simulink model "bins_model2"  (Simulink 8.3)
settings: Solver=ode45  StartTime=0.0  StopTime=300  MaxStep=0.1  RelTol=1e-3
libraries: aerolibnav x1
settings Model: Creator=me  LastModifiedBy=me
settings DataIOCC: SignalLoggingSaveFormat=Dataset
settings DebuggingCC: UnderspecifiedInitializationDetection=Simplified  StateNameClashWarn=none
settings GRTTargetCC: CombineOutputUpdateFcns=on  GRTInterface=off

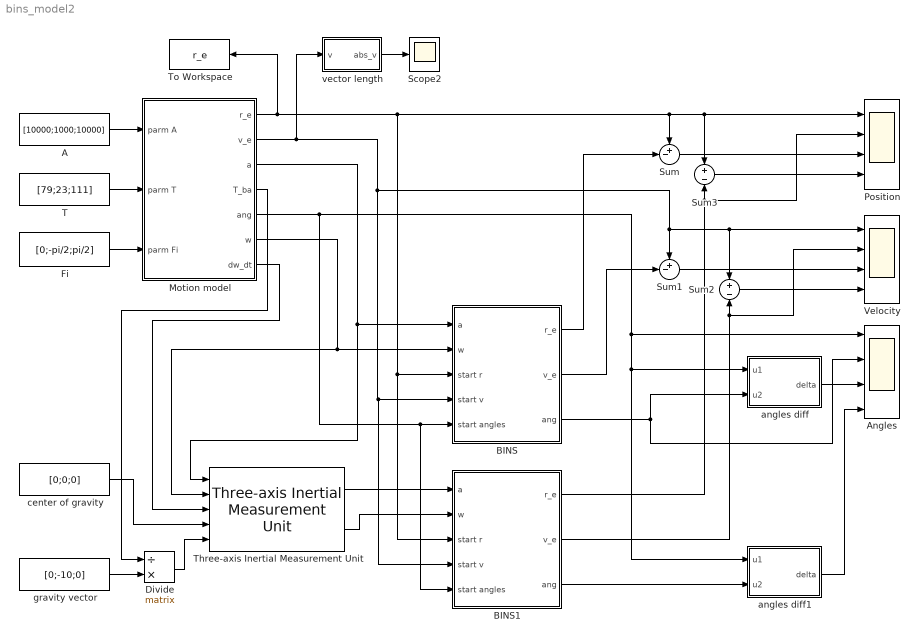
== system bins_model2 ==
  A : Constant  Value=[10000;1000;10000]
  Angles : Scope  NumInputPorts=4
      settings: TimeRange=300  YMin=-4~-4~-3e-15~-7  YMax=4~4~4e-15~1  SaveName=ScopeData3  MaxDataPoints=200000
  BINS : Subsystem
  BINS1 : Subsystem
  Divide : Product  Inputs=/*  Multiplication=Matrix(*)
  Fi : Constant  Value=[0;-pi/2;pi/2]
  Motion model : Subsystem
  Position : Scope  NumInputPorts=4
      settings: TimeRange=300  YMin=-10000~-20000~-1e-09~-10000  YMax=10000~20000~3e-09~5000  MaxDataPoints=200000
  Scope2 : Scope
      settings: TimeRange=1000  YMin=0  YMax=1000  SaveName=ScopeData2  MaxDataPoints=50000
  Sum : Sum  Inputs=+-|
  Sum1 : Sum  Inputs=+-|
  Sum2 : Sum  Inputs=+-
  Sum3 : Sum  Inputs=+-
  T : Constant  Value=[79;23;111]
  Three-axis Inertial Measurement Unit : aerolibnav/Three-axis Inertial Measurement Unit  units=Metric (MKS)  imu=[0 0 0]  dtype_a=off  w_a=190  z_a=0.707  a_sf_cc=[1 0 0; 0 1 0; 0 0 1]  a_bias=[0 0 0]  a_sat="[-inf  -inf  -inf  inf inf inf]"  dtype_g=off  w_g=190  z_g=0.707  g_sf_cc=[1 0 0; 0 1 0; 0 0 1]  g_bias=[0 0 0]  g_sens=[0 0 0]  g_sat="[-inf  -inf  -inf  inf inf inf]"  i_rand=on  i_seeds=[23093 23094 23095 23096 23097 23098]  i_pow=[0.0001 0.0001 0.0001 0.000001 0.000001 0.000001]  i_Ts=0
  To Workspace : ToWorkspace  VariableName=r_e  SaveFormat=Timeseries  SampleTime=-1
  Velocity : Scope  NumInputPorts=4
      settings: TimeRange=1000  YMin=-1000~-1000~-1e-09~-100  YMax=1000~1000~1e-09~100  SaveName=ScopeData4  MaxDataPoints=200000
  angles diff : MATLAB Function  TreatAsAtomicUnit=on
  angles diff1 : MATLAB Function  TreatAsAtomicUnit=on
  center of gravity : Constant  Value=[0;0;0]
  gravity vector : Constant  Value=[0;-10;0]
  vector length : Subsystem
  wires:
  vector length/1(abs_v) -> Scope2/1
  A/1 -> Motion model/1(parm A)
  T/1 -> Motion model/2(parm T)
  Fi/1 -> Motion model/3(parm Fi)
  Motion model/1(r_e) -> BINS1/3(start r), BINS/3(start r), Sum/1, Position/1, Sum3/1, To Workspace/1
  Motion model/5(ang) -> BINS1/5(start angles), BINS/5(start angles), angles diff1/1(u1), angles diff/1(u1), Angles/1
  Motion model/3(a) -> Three-axis Inertial Measurement Unit/1, BINS/1(a)
  Motion model/7(dw_dt) -> Three-axis Inertial Measurement Unit/3
  BINS/3(ang) -> angles diff/2(u2), Angles/2
  angles diff/1(delta) -> Angles/3
  BINS/1(r_e) -> Sum/2
  Sum/1 -> Position/3
  Motion model/2(v_e) -> BINS1/4(start v), BINS/4(start v), Sum1/1, Sum2/1, Velocity/1, vector length/1(v)
  BINS/2(v_e) -> Sum1/2
  Sum1/1 -> Velocity/3
  center of gravity/1 -> Three-axis Inertial Measurement Unit/4
  Three-axis Inertial Measurement Unit/1 -> BINS1/1(a)
  Three-axis Inertial Measurement Unit/2 -> BINS1/2("w ")
  Motion model/6(w) -> Three-axis Inertial Measurement Unit/2, BINS/2("w ")
  BINS1/3(ang) -> angles diff1/2(u2)
  angles diff1/1(delta) -> Angles/4
  Sum2/1 -> Velocity/4
  Sum3/1 -> Position/4
  BINS1/1(r_e) -> Position/2, Sum3/2
  BINS1/2(v_e) -> Velocity/2, Sum2/2
  gravity vector/1 -> Divide/2
  Divide/1 -> Three-axis Inertial Measurement Unit/5
  Motion model/4(T_ba) -> Divide/1

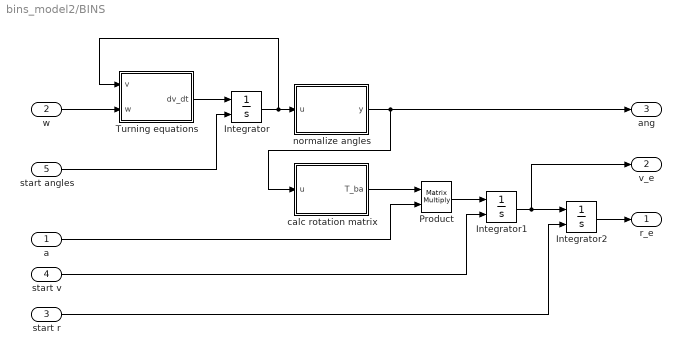
== system bins_model2/BINS ==
  a : Inport
  "w " : Inport  Port=2
  start r : Inport  Port=3
  start v : Inport  Port=4
  start angles : Inport  Port=5
  Integrator : Integrator  InitialConditionSource=external
  Integrator1 : Integrator  InitialConditionSource=external
  Integrator2 : Integrator  InitialConditionSource=external
  Product : Product  Multiplication=Matrix(*)
  Turning equations : MATLAB Function  TreatAsAtomicUnit=on
  calc rotation matrix : MATLAB Function  TreatAsAtomicUnit=on
  normalize angles : MATLAB Function  TreatAsAtomicUnit=on
  r_e : Outport
  v_e : Outport  Port=2
  ang : Outport  Port=3
  wires:
  Product/1 -> Integrator1/1
  Turning equations/1(dv_dt) -> Integrator/1
  Integrator/1 -> Turning equations/1(v), normalize angles/1(u)
  normalize angles/1(y) -> calc rotation matrix/1(u), ang/1
  Integrator1/1 -> Integrator2/1, v_e/1
  start r/1 -> Integrator2/2
  a/1 -> Product/2
  start v/1 -> Integrator1/2
  start angles/1 -> Integrator/2
  calc rotation matrix/1(T_ba) -> Product/1
  Integrator2/1 -> r_e/1
  "w "/1 -> Turning equations/2(w)

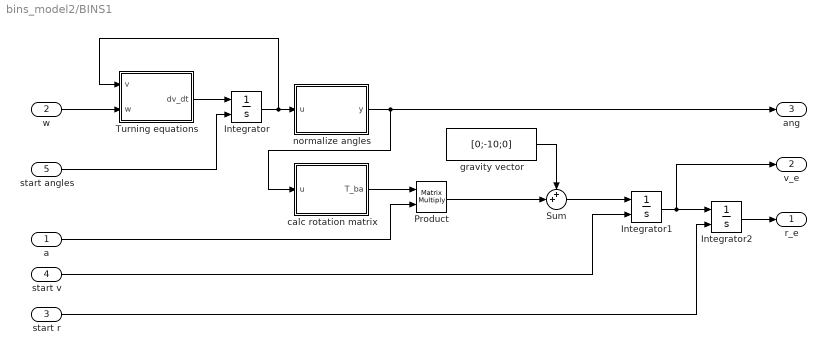
== system bins_model2/BINS1 ==
  a : Inport
  "w " : Inport  Port=2
  start r : Inport  Port=3
  start v : Inport  Port=4
  start angles : Inport  Port=5
  Integrator : Integrator  InitialConditionSource=external
  Integrator1 : Integrator  InitialConditionSource=external
  Integrator2 : Integrator  InitialConditionSource=external
  Product : Product  Multiplication=Matrix(*)
  Sum : Sum  Inputs=++|
  Turning equations : MATLAB Function  TreatAsAtomicUnit=on
  calc rotation matrix : MATLAB Function  TreatAsAtomicUnit=on
  gravity vector : Constant  Value=[0;-10;0]
  normalize angles : MATLAB Function  TreatAsAtomicUnit=on
  r_e : Outport
  v_e : Outport  Port=2
  ang : Outport  Port=3
  wires:
  Turning equations/1(dv_dt) -> Integrator/1
  Integrator/1 -> Turning equations/1(v), normalize angles/1(u)
  normalize angles/1(y) -> calc rotation matrix/1(u), ang/1
  Integrator1/1 -> Integrator2/1, v_e/1
  start r/1 -> Integrator2/2
  a/1 -> Product/2
  start angles/1 -> Integrator/2
  calc rotation matrix/1(T_ba) -> Product/1
  Integrator2/1 -> r_e/1
  "w "/1 -> Turning equations/2(w)
  gravity vector/1 -> Sum/1
  Sum/1 -> Integrator1/1
  Product/1 -> Sum/2
  start v/1 -> Integrator1/2

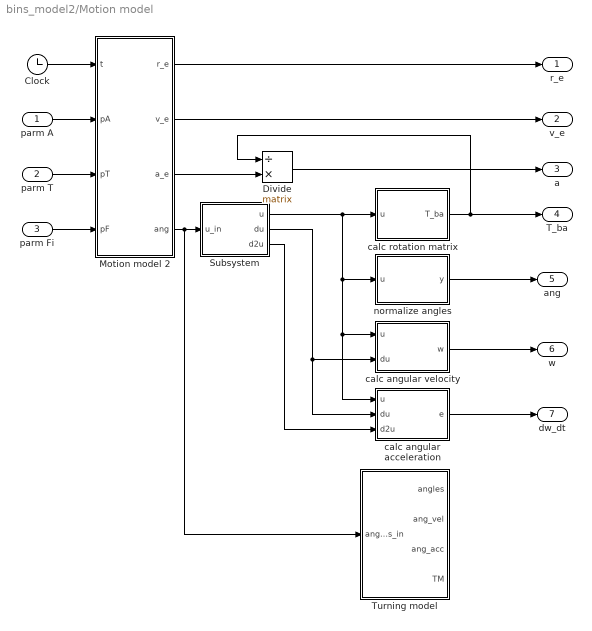
== system bins_model2/Motion model ==
  parm A : Inport
  parm T : Inport  Port=2
  parm Fi : Inport  Port=3
  Clock : Clock
  Divide : Product  Inputs=/*  Multiplication=Matrix(*)
  Motion model 2 : MATLAB Function  TreatAsAtomicUnit=on
  Subsystem : Subsystem
  Turning model : Subsystem
  calc angular acceleration : MATLAB Function  TreatAsAtomicUnit=on
  calc angular velocity : MATLAB Function  TreatAsAtomicUnit=on
  calc rotation matrix : MATLAB Function  TreatAsAtomicUnit=on
  normalize angles : MATLAB Function  TreatAsAtomicUnit=on
  r_e : Outport
  v_e : Outport  Port=2
  a : Outport  Port=3
  T_ba : Outport  Port=4
  ang : Outport  Port=5
  w : Outport  Port=6
  dw_dt : Outport  Port=7
  wires:
  parm Fi/1 -> Motion model 2/4(pF)
  parm A/1 -> Motion model 2/2(pA)
  parm T/1 -> Motion model 2/3(pT)
  Subsystem/2(du) -> calc angular acceleration/2(du), calc angular velocity/2(du)
  Subsystem/1(u) -> calc angular acceleration/1(u), calc angular velocity/1(u), normalize angles/1(u), calc rotation matrix/1(u)
  Motion model 2/4(ang) -> Turning model/1(angles_in), Subsystem/1(u_in)
  Motion model 2/1(r_e) -> r_e/1
  calc angular acceleration/1(e) -> dw_dt/1
  Subsystem/3(d2u) -> calc angular acceleration/3(d2u)
  calc angular velocity/1(w) -> w/1
  Motion model 2/2(v_e) -> v_e/1
  Motion model 2/3(a_e) -> Divide/2
  Clock/1 -> Motion model 2/1(t)
  normalize angles/1(y) -> ang/1
  calc rotation matrix/1(T_ba) -> T_ba/1, Divide/1
  Divide/1 -> a/1

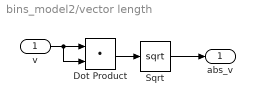
== system bins_model2/vector length ==
  v : Inport
  Dot Product : DotProduct  InputSameDT=on  OutDataTypeStr=Inherit: Inherit via internal rule
  Sqrt : Sqrt  SaturateOnIntegerOverflow=on
  abs_v : Outport
  wires:
  Sqrt/1 -> abs_v/1
  Dot Product/1 -> Sqrt/1
  v/1 -> Dot Product/2, Dot Product/1

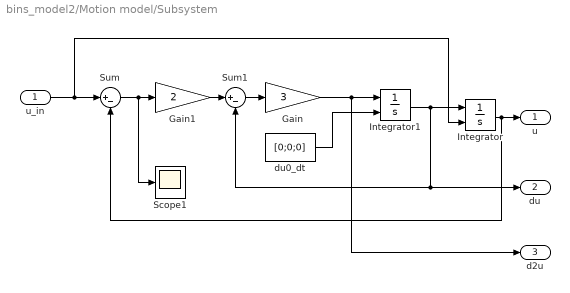
== system bins_model2/Motion model/Subsystem ==
  u_in : Inport
  Gain : Gain  Gain=3
  Gain1 : Gain  Gain=2
  Integrator : Integrator  InitialConditionSource=external
  Integrator1 : Integrator  InitialConditionSource=external
  Scope1 : Scope
      settings: YMin=-1.5  YMax=0.1
  Sum : Sum  Inputs=|+-
  Sum1 : Sum  Inputs=|+-
  du0_dt : Constant  Value=[0;0;0]
  u : Outport
  du : Outport  Port=2
  d2u : Outport  Port=3
  wires:
  Sum1/1 -> Gain/1
  Gain1/1 -> Sum1/1
  Integrator/1 -> u/1, Sum/2
  Sum/1 -> Gain1/1, Scope1/1
  Gain/1 -> d2u/1, Integrator1/1
  du0_dt/1 -> Integrator1/2
  Integrator1/1 -> Integrator/1, Sum1/2, du/1
  u_in/1 -> Integrator/2, Sum/1

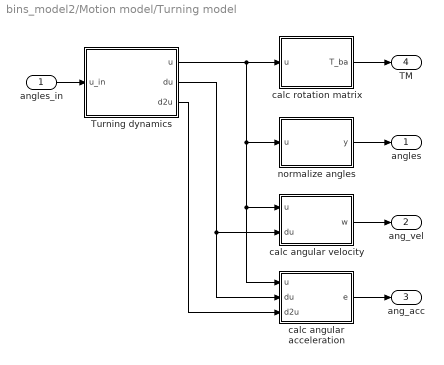
== system bins_model2/Motion model/Turning model ==
  angles_in : Inport
  Turning dynamics : Subsystem
  calc angular acceleration : MATLAB Function  TreatAsAtomicUnit=on
  calc angular velocity : MATLAB Function  TreatAsAtomicUnit=on
  calc rotation matrix : MATLAB Function  TreatAsAtomicUnit=on
  normalize angles : MATLAB Function  TreatAsAtomicUnit=on
  angles : Outport
  ang_vel : Outport  Port=2
  ang_acc : Outport  Port=3
  TM : Outport  Port=4
  wires:
  Turning dynamics/2(du) -> calc angular acceleration/2(du), calc angular velocity/2(du)
  Turning dynamics/1(u) -> calc angular acceleration/1(u), calc angular velocity/1(u), normalize angles/1(u), calc rotation matrix/1(u)
  calc angular acceleration/1(e) -> ang_acc/1
  Turning dynamics/3(d2u) -> calc angular acceleration/3(d2u)
  calc angular velocity/1(w) -> ang_vel/1
  normalize angles/1(y) -> angles/1
  calc rotation matrix/1(T_ba) -> TM/1
  angles_in/1 -> Turning dynamics/1(u_in)

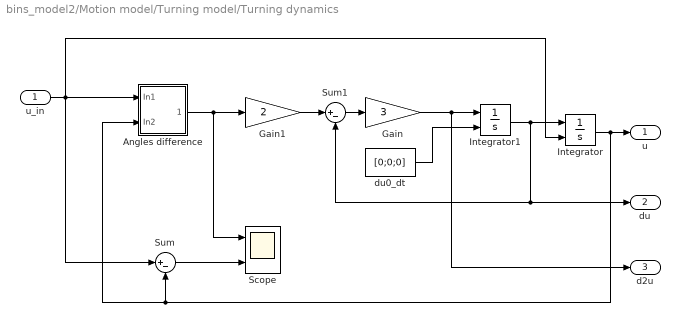
== system bins_model2/Motion model/Turning model/Turning dynamics ==
  u_in : Inport
  Angles difference : Subsystem
  Gain : Gain  Gain=3
  Gain1 : Gain  Gain=2
  Integrator : Integrator  InitialConditionSource=external
  Integrator1 : Integrator  InitialConditionSource=external
  Scope : Scope  NumInputPorts=2
      settings: YMin=-1.5~-3.5  YMax=6.5~3.5  SaveName=ScopeData10  MaxDataPoints=50000
  Sum : Sum  Inputs=|+-
  Sum1 : Sum  Inputs=|+-
  du0_dt : Constant  Value=[0;0;0]
  u : Outport
  du : Outport  Port=2
  d2u : Outport  Port=3
  wires:
  Sum1/1 -> Gain/1
  Gain1/1 -> Sum1/1
  Gain/1 -> d2u/1, Integrator1/1
  du0_dt/1 -> Integrator1/2
  Integrator1/1 -> Integrator/1, Sum1/2, du/1
  u_in/1 -> Sum/1, Integrator/2, Angles difference/1(In1)
  Integrator/1 -> Angles difference/2(In2), Sum/2, u/1
  Angles difference/1(Out1) -> Gain1/1, Scope/1
  Sum/1 -> Scope/2

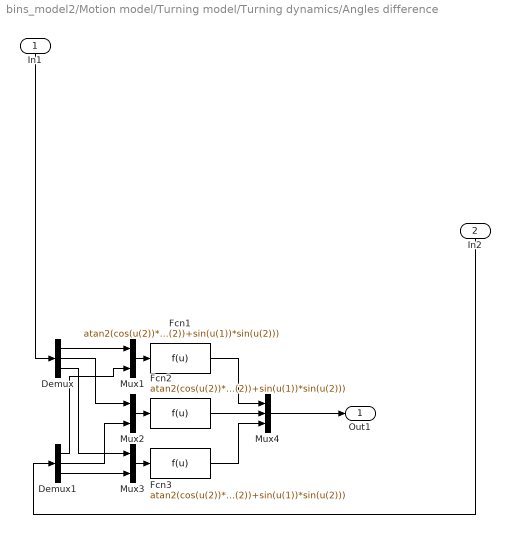
== system bins_model2/Motion model/Turning model/Turning dynamics/Angles difference ==
  In1 : Inport
  In2 : Inport  Port=2
  Demux : Demux  Outputs=3
  Demux1 : Demux  Outputs=3
  Fcn1 : Fcn  Expr=atan2(cos(u(2))*sin(u(1))-sin(u(2))*cos(u(1)),cos(u(1))*cos(u(2))+sin(u(1))*sin(u(2)))
  Fcn2 : Fcn  Expr=atan2(cos(u(2))*sin(u(1))-sin(u(2))*cos(u(1)),cos(u(1))*cos(u(2))+sin(u(1))*sin(u(2)))
  Fcn3 : Fcn  Expr=atan2(cos(u(2))*sin(u(1))-sin(u(2))*cos(u(1)),cos(u(1))*cos(u(2))+sin(u(1))*sin(u(2)))
  Mux1 : Mux  Inputs=2
  Mux2 : Mux  Inputs=2
  Mux3 : Mux  Inputs=2
  Mux4 : Mux  Inputs=3
  Out1 : Outport
  wires:
  In2/1 -> Demux1/1
  In1/1 -> Demux/1
  Mux2/1 -> Fcn2/1
  Demux/1 -> Mux1/1
  Demux1/2 -> Mux2/2
  Mux4/1 -> Out1/1
  Demux/2 -> Mux2/1
  Fcn1/1 -> Mux4/1
  Fcn2/1 -> Mux4/2
  Demux/3 -> Mux3/1
  Demux1/1 -> Mux1/2
  Demux1/3 -> Mux3/2
  Fcn3/1 -> Mux4/3
  Mux3/1 -> Fcn3/1
  Mux1/1 -> Fcn1/1

== matlab function Motion model/Motion model 2 ==
  data: t input double; r_e output double; pA input double; pT input double; pF input double; v_e output double; a_e output double; ang output double
function [r_e, v_e, a_e, ang] = fcn(t, pA, pT, pF)
%#codegen

    [r_e, v_e, a_e, ~, ang] = f_motion_model2(t, pA, pT, pF);

end

== matlab function Motion model/calc angular velocity ==
  data: u input double; w output double; du input double
function w = fcn(u, du)
%#codegen

w = f_calc_ang_vel(u, du);

== matlab function Motion model/normalize angles ==
  data: u input double; y output double
function y = fcn(u)
%#codegen
y = u;
for i=1:length(y)
    y(i)=f_normalize_angle(u(i));
end

== matlab function Motion model/calc angular acceleration ==
  data: u input double; e output double; du input double; d2u input double
function e = fcn(u, du, d2u)
%#codegen

e = f_calc_ang_accel(u, du, d2u);

== matlab function Motion model/calc rotation matrix ==
  data: u input double; T_ba output double
function T_ba = fcn(u)
%#codegen

T_ba = f_calc_turn_matrix_from_angles(u);

== matlab function BINS/Turning equations ==
  data: v input double; dv_dt output double; w input double
function dv_dt = fcn(v, w)
%#codegen

    dv_dt = f_turning_by_Euler(v, w);
    
end

== matlab function BINS/normalize angles ==
  data: u input double; y output double
function y = fcn(u)
%#codegen
y = u;
for i=1:length(y)
    y(i)=f_normalize_angle(u(i));
end

== matlab function BINS/calc rotation matrix ==
  data: u input double; T_ba output double
function T_ba = fcn(u)
%#codegen

T_ba = f_calc_turn_matrix_from_angles(u);

== matlab function angles diff ==
  data: u1 input double; delta output double; u2 input double
function delta = fcn(u1, u2)
%#codegen

delta = f_angles_diff(u1,u2);

end

== matlab function BINS1/Turning equations ==
  data: v input double; dv_dt output double; w input double
function dv_dt = fcn(v, w)
%#codegen

    dv_dt = f_turning_by_Euler(v, w);
    
end

== matlab function BINS1/calc rotation matrix ==
  data: u input double; T_ba output double
function T_ba = fcn(u)
%#codegen

T_ba = f_calc_turn_matrix_from_angles(u);

== matlab function BINS1/normalize angles ==
  data: u input double; y output double
function y = fcn(u)
%#codegen
y = u;
for i=1:length(y)
    y(i)=f_normalize_angle(u(i));
end

== matlab function angles diff1 ==
  data: u1 input double; delta output double; u2 input double
function delta = fcn(u1, u2)
%#codegen

delta = f_angles_diff(u1,u2);

end

== matlab function Motion model/Turning model/calc angular acceleration ==
  data: u input double; e output double; du input double; d2u input double
function e = fcn(u, du, d2u)
%#codegen

e = f_calc_ang_accel(u, du, d2u);

== matlab function Motion model/Turning model/calc angular velocity ==
  data: u input double; w output double; du input double
function w = fcn(u, du)
%#codegen

w = f_calc_ang_vel(u, du);

== matlab function Motion model/Turning model/calc rotation matrix ==
  data: u input double; T_ba output double
function T_ba = fcn(u)
%#codegen

T_ba = f_calc_turn_matrix_from_angles(u);

== matlab function Motion model/Turning model/normalize angles ==
  data: u input double; y output double
function y = fcn(u)
%#codegen
y = u;
for i=1:length(y)
    y(i)=f_normalize_angle(u(i));
end
